simulink model "v1_2025_10_20_D1_first_team_draft"  (R2025a)
settings: Solver=FixedStepAuto  StartTime=0.0  StopTime=10.0  FixedStep=1e-3  RelTol=1e-3  EnableMultiTasking=on
undefined symbols (not defined in the file): D0, D1, D10, D11, D12, D13, D2, D3, D4, D5, D6, D7, D8, D9, PTA0, PTA1, PTA2, PTB23, PTB9, PTC16, PTC17, PTC2, PTC3, PTC4, PTD0, PTD1, PTD2, PTD3
libraries: frdmk64flib x14
settings Model: ExtModeTrigDuration=5  Creator=seohj  LastModifiedBy=seohj
settings OptimizationCC: DefaultParameterBehavior=Inlined  EnhancedBackFolding=on  PassReuseOutputArgsAs=Individual arguments  ZeroExternalMemoryAtStartup=off  ZeroInternalMemoryAtStartup=off  MaxStackSize=64  OptimizeBlockOrder=speed  DifferentSizesBufferReuse=on  OptimizationCustomize=off  EfficientTunableParamExpr=on
settings DebuggingCC: ParameterTunabilityLossMsg=error
settings HardwareCC: ProdBitPerPointer=32.0  ProdBitPerSizeT=32.0  ProdBitPerPtrDiffT=32.0  ProdLargestAtomicInteger=Long  ProdLargestAtomicFloat=Double  ProdWordSize=32.0  ProdHWDeviceType=ARM Compatible->ARM Cortex
settings SFSimCC: MATLABDynamicMemAlloc=off
settings RTWCC: SystemTargetFile=ert.tlc  HardwareBoard=NXP FRDM-K64F  TLCOptions="-aInlineSetEventsForThisBaseRateFcn=TLC_FALSE -aSuppressMultiTaskScheduler=TLC_FALSE  -aRateBasedStepFcn=0"  TemplateMakefile=ert_default_tmf  Toolchain=GNU Tools for ARM Embedded Processors  Description=Embedded Coder
settings CodeAppCC: ForceParamTrailComments=on  IgnoreCustomStorageClasses=off  OperatorAnnotations=on  SimulinkDataObjDesc=on  SFDataObjDesc=on  InsertBlockDesc=on
settings ERTTargetCC: ExtModeTransport=4.0  ExtModeStaticAlloc=off  ExtModeMexFile=sendToCommService  ExtModeIntrfLevel=Level1

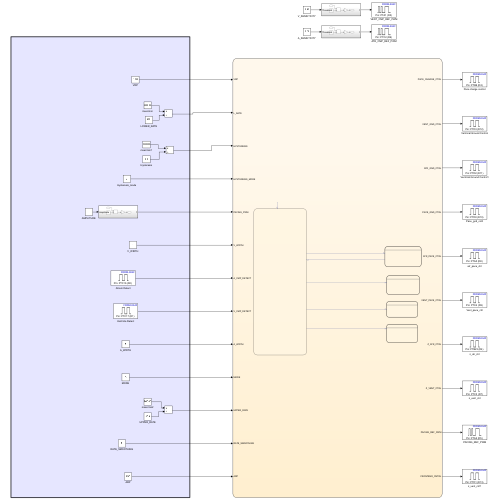
[thumbnail: Simulink's stored preview of the top-level diagram]
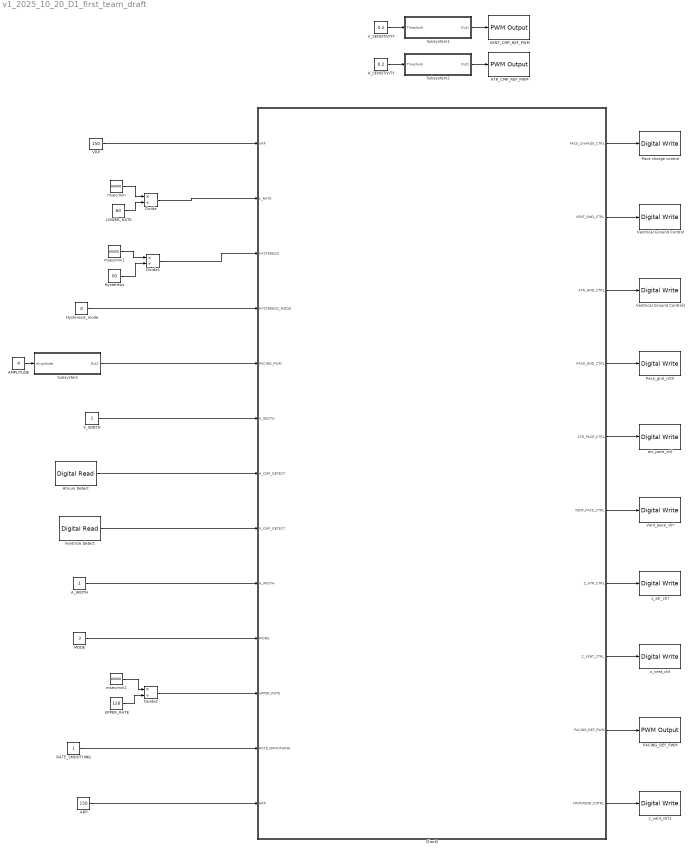
== system v1_2025_10_20_D1_first_team_draft ==
  AMPLITUDE : Constant  Value=4  OutDataTypeStr=int16
  ARP : Constant  Value=150  OutDataTypeStr=int16
  ATR_CMP_REF_PWM : frdmk64flib/PWM Output  Whichpin=PTC2 (D6)  InitialFrequency=2000  InitialDutyCycle=0
  A_SENSITIVITY : Constant  Value=0.2  OutDataTypeStr=double
  A_WIDTH : Constant  OutDataTypeStr=int16
  Atrium Detect : frdmk64flib/Digital Read  Whichpin=PTC16 (D0)  SampleTime=-1
  Chart2 : Stateflow chart  TreatAsAtomicUnit=on
      settings: PortSchema="{\"entries\":[{\"content\":{\"sides\":[{\"content\":{\"connectorIds\":[\"In1\",\"In8\",\"In3\",\"In4\",\"In5\",\"In9\",\"In10\",\"In11\",\"In12\",\"In6\",\"In13\",\"In7\",\"In2\"]},\"type\":\"ConnectorPlacement.EquallySpacedRectSide\",\"uuid\":\"eb0c691f-8d42-442e-bcbf-fb5e5d0eed13\"},{\"content\":{\"connectorIds\":[\"Out1\",\"Out2\",\"Out3\",\"Out4\",\"Out5\",\"Out6\",\"Out7\",\"Out8\",\"Out9\",\"Out10\"],\"side\":\"RIGHT\"},\"type\":\"ConnectorPlacement.EquallySpacedRectSide\",\"uuid\":\"51fddc5a-1884-4d13-98b7-b2e7f62644c5\"},{\"content\":{\"side\":\"TOP\"},\"type\":\"ConnectorPlacement.EquallySpacedRectSide\",\"uuid\":\"c0de6dfc-3a40-48f1-a3e4-7cd76d4b9b4b\"},{\"content\":{\"side\":\"BOTTOM\"},\"type\":\"ConnectorPlacement.EquallySpacedRectSide\",\"uuid\":\"2c1acec7-1ddf-4f64-9578-e80022136ca6\"}]},\"type\":\"ConnectorPlacement.EquallySpacedConnector\",\"uuid\":\"3f5ef44b-ad1c-43dd-8b19-21cef7f1f7f1\"}],\"packageUris\":[\"http://schema.mathworks.com/mf0/Connector/R2020b\"],\"version\":\"1.0\"}"
  Divide : Product  Inputs=*/
  Divide1 : Product  Inputs=*/
  Divide2 : Product  Inputs=*/
  Hysteresis : Constant  Value=50
  Hysteresis_mode : Constant  Value=0
  LOWER_RATE : Constant  Value=60  OutDataTypeStr=int16
  MODE : Constant  Value=3  OutDataTypeStr=int16
  PACING_REF_PWM : frdmk64flib/PWM Output  Whichpin=PTA2 (D5)  InitialFrequency=2000  InitialDutyCycle=0
  Pace charge control : frdmk64flib/Digital Write  Whichpin=PTB9 (D2)
  Pace_gnd_cntrl : frdmk64flib/Digital Write  Whichpin=PTD0 (D10)
  RATE_SMOOTHING : Constant  OutDataTypeStr=int16
  Subsystem : Subsystem
  Subsystem1 : Subsystem
  Subsystem2 : Subsystem
  UPPER_RATE : Constant  Value=128  OutDataTypeStr=int16
  VENT_CMP_REF_PWM : frdmk64flib/PWM Output  Whichpin=PTA1 (D3)  InitialFrequency=2000  InitialDutyCycle=0
  VRP : Constant  Value=150  OutDataTypeStr=int16
  V_SENSITIVITY : Constant  Value=0.2  OutDataTypeStr=double
  V_WIDTH : Constant  OutDataTypeStr=int16
  Vent_pace_ctrl : frdmk64flib/Digital Write  Whichpin=PTC4 (D9)
  Ventrical Ground Control : frdmk64flib/Digital Write  Whichpin=PTD3 (D12)
  Ventrical Ground Control1 : frdmk64flib/Digital Write  Whichpin=PTD2 (D11)
  Ventricle Detect : frdmk64flib/Digital Read  Whichpin=PTC17 (D1)  SampleTime=-1
  atr_pace_ctrl : frdmk64flib/Digital Write  Whichpin=PTA0 (D8)
  msec/min : Constant  Value=60000  OutDataTypeStr=double  LockScale=on
  msec/min1 : Constant  Value=60000  OutDataTypeStr=double  LockScale=on
  msec/min2 : Constant  Value=60000  OutDataTypeStr=double  LockScale=on
  z_atr_ctrl : frdmk64flib/Digital Write  Whichpin=PTB23 (D4)
  z_vent_ctrl : frdmk64flib/Digital Write  Whichpin=PTC3 (D7)
  z_vent_ctrl1 : frdmk64flib/Digital Write  Whichpin=PTD1 (D13)
  wires:
  A_WIDTH/1 -> Chart2/12(A_WIDTH)
  V_WIDTH/1 -> Chart2/9(V_WIDTH)
  Ventricle Detect/1 -> Chart2/11(V_CMP_DETECT)
  RATE_SMOOTHING/1 -> Chart2/7(RATE_SMOOTHING)
  VRP/1 -> Chart2/1(VRP)
  ARP/1 -> Chart2/2(ARP)
  MODE/1 -> Chart2/6(MODE)
  Atrium Detect/1 -> Chart2/10(A_CMP_DETECT)
  msec/min/1 -> Divide/1
  LOWER_RATE/1 -> Divide/2
  Divide/1 -> Chart2/8(L_RATE)
  msec/min1/1 -> Divide1/1
  Divide1/1 -> Chart2/3(HYSTERESIS)
  msec/min2/1 -> Divide2/1
  Divide2/1 -> Chart2/13(UPPER_RATE)
  UPPER_RATE/1 -> Divide2/2
  Chart2/1(PACE_CHARGE_CTRL) -> Pace charge control/1
  Chart2/2(VENT_GND_CTRL) -> Ventrical Ground Control/1
  Chart2/3(ATR_GND_CTRL) -> Ventrical Ground Control1/1
  Chart2/7(Z_ATR_CTRL) -> z_atr_ctrl/1
  Chart2/8(Z_VENT_CTRL) -> z_vent_ctrl/1
  Chart2/6(VENT_PACE_CTRL) -> Vent_pace_ctrl/1
  Chart2/5(ATR_PACE_CTRL) -> atr_pace_ctrl/1
  Chart2/4(PACE_GND_CTRL) -> Pace_gnd_cntrl/1
  Chart2/9(PACING_REF_PWM) -> PACING_REF_PWM/1
  AMPLITUDE/1 -> Subsystem/1(Amplitude)
  Subsystem/1(Out1) -> Chart2/5(PACING_PWM)
  Subsystem1/1(Out1) -> VENT_CMP_REF_PWM/1
  V_SENSITIVITY/1 -> Subsystem1/1(Threshold)
  Subsystem2/1(Out1) -> ATR_CMP_REF_PWM/1
  A_SENSITIVITY/1 -> Subsystem2/1(Threshold)
  Hysteresis/1 -> Divide1/2
  Hysteresis_mode/1 -> Chart2/4(HYSTERESIS_MODE)
  Chart2/10(FRONTEND_CNTRL) -> z_vent_ctrl1/1

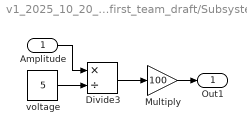
== system v1_2025_10_20_D1_first_team_draft/Subsystem ==
  Amplitude : Inport
  Divide3 : Product  Inputs=*/
  Multiply : Gain  Gain=100
  voltage : Constant  Value=5  OutDataTypeStr=int16
  Out1 : Outport
  wires:
  Divide3/1 -> Multiply/1
  Multiply/1 -> Out1/1
  voltage/1 -> Divide3/2
  Amplitude/1 -> Divide3/1

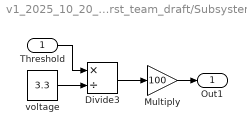
== system v1_2025_10_20_D1_first_team_draft/Subsystem1 ==
  Threshold : Inport
  Divide3 : Product  Inputs=*/
  Multiply : Gain  Gain=100
  voltage : Constant  Value=3.3  OutDataTypeStr=double
  Out1 : Outport
  wires:
  Divide3/1 -> Multiply/1
  Multiply/1 -> Out1/1
  voltage/1 -> Divide3/2
  Threshold/1 -> Divide3/1

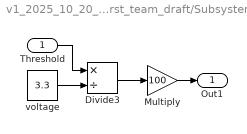
== system v1_2025_10_20_D1_first_team_draft/Subsystem2 ==
  Threshold : Inport
  Divide3 : Product  Inputs=*/
  Multiply : Gain  Gain=100
  voltage : Constant  Value=3.3  OutDataTypeStr=double
  Out1 : Outport
  wires:
  Divide3/1 -> Multiply/1
  Multiply/1 -> Out1/1
  voltage/1 -> Divide3/2
  Threshold/1 -> Divide3/1

== stateflow chart v1_2025_10_20_D1_first_team_draft/Chart2 ==
  state START
  state AOO
    state AOO
      entry:
      %Charge Capacitor
      PACING_REF_PWM = PACING_PWM
      ATR_PACE_CTRL = LOW
      VENT_PACE_CTRL = LOW
      PACE_CHARGE_CTRL = HIGH
      %Discharge Blocking Capactior
      PACE_GND_CTRL = HIGH
      VENT_PACE_CTRL = LOW
      Z_ATR_CTRL = LOW
      Z_VENT_CTRL = LOW
      ATR_PACE_CTRL = LOW
      ATR_GND_CTRL = HIGH
      VENT_GND_CTRL = LOW
    state AOO_PULSE
      entry:
      %Begin discharging C22 and charging C21
      PACE_CHARGE_CTRL= LOW
      PACE_GND_CTRL = HIGH
      ATR_PACE_CTRL = HIGH
      ATR_GND_CTRL = LOW
      Z_ATR_CTRL = LOW
      Z_VENT_CTRL = LOW
      VENT_GND_CTRL = LOW
      VENT_PACE_CTRL = LOW
    (default) -> AOO.AOO
    AOO.AOO -> AOO_PULSE : [after(L_RATE - A_WIDTH,msec)]
    AOO_PULSE -> AOO.AOO : [after(A_WIDTH,msec)]
  state VOO
    state VOO
      entry:
      %Charge Capacitor C22
      ATR_PACE_CTRL = LOW
      VENT_PACE_CTRL = LOW
      PACING_REF_PWM = PACING_PWM
      PACE_CHARGE_CTRL = HIGH
      %Discharge Blocking Capacitor
      VENT_PACE_CTRL = LOW
      PACE_GND_CTRL = HIGH
      ATR_PACE_CTRL = LOW
      ATR_GND_CTRL = LOW
      Z_ATR_CTRL = LOW
      Z_VENT_CTRL = LOW
      VENT_GND_CTRL = HIGH
    state VOO_PULSE
      entry:
      %Begin discharging C22 and charging C21
      PACE_CHARGE_CTRL= LOW
      PACE_GND_CTRL = HIGH
      ATR_PACE_CTRL = LOW
      ATR_GND_CTRL = LOW
      Z_ATR_CTRL = LOW
      Z_VENT_CTRL = LOW
      VENT_GND_CTRL = LOW
      VENT_PACE_CTRL = HIGH
    (default) -> VOO.VOO
    VOO.VOO -> VOO_PULSE : [after(L_RATE - V_WIDTH,msec)]
    VOO_PULSE -> VOO.VOO : [after(V_WIDTH,msec)]
  state AAI
    state AAI
      entry:
      %Charge Capacitor
      PACING_REF_PWM = PACING_PWM
      ATR_PACE_CTRL = LOW
      VENT_PACE_CTRL = LOW
      PACE_CHARGE_CTRL = HIGH
      %Discharge Blocking Capactior
      PACE_GND_CTRL = HIGH
      VENT_PACE_CTRL = LOW
      Z_ATR_CTRL = LOW
      Z_VENT_CTRL = LOW
      ATR_PACE_CTRL = LOW
      ATR_GND_CTRL = HIGH
      VENT_GND_CTRL = LOW
      FRONTEND_CNTRL = HIGH
    state AAI_PULSE
      entry:
      %Begin discharging C22 and charging C21
      PACE_CHARGE_CTRL= LOW
      PACE_GND_CTRL = HIGH
      ATR_PACE_CTRL = HIGH
      ATR_GND_CTRL = LOW
      Z_ATR_CTRL = LOW
      Z_VENT_CTRL = LOW
      VENT_GND_CTRL = LOW
      VENT_PACE_CTRL = LOW
      FRONTEND_CNTRL = LOW
    state Buffer
    state AAI_ARP
      entry:
      %Charge Capacitor
      PACING_REF_PWM = PACING_PWM
      ATR_PACE_CTRL = LOW
      VENT_PACE_CTRL = LOW
      PACE_CHARGE_CTRL = LOW
      %Discharge Blocking Capactior
      PACE_GND_CTRL = HIGH
      VENT_PACE_CTRL = LOW
      Z_ATR_CTRL = LOW
      Z_VENT_CTRL = LOW
      ATR_PACE_CTRL = LOW
      ATR_GND_CTRL = HIGH
      VENT_GND_CTRL = LOW
      FRONTEND_CNTRL = LOW
    AAI.AAI -> AAI_PULSE [order 2] : [after(HYSTERESIS - A_WIDTH-ARP,msec) & HYSTERESIS_MODE == 1]
    (default) -> AAI.AAI
    AAI.AAI -> AAI_PULSE [order 3] : [after(L_RATE - A_WIDTH-ARP,msec) & HYSTERESIS_MODE == 0 ]
    AAI.Buffer -> AAI.Buffer [order 2] : [A_CMP_DETECT == HIGH]
    AAI.AAI -> AAI.Buffer [order 1] : [A_CMP_DETECT == HIGH]
    AAI.Buffer -> AAI.AAI [order 3] : [after(HYSTERESIS,msec) & HYSTERESIS_MODE ==1]
    AAI.Buffer -> AAI.AAI [order 1] : [after(L_RATE,msec) & HYSTERESIS_MODE == 0]
    AAI_PULSE -> AAI_ARP : [after(A_WIDTH,msec)]
    AAI_ARP -> AAI.AAI : [after(ARP,msec)]
  state VVI
    state VVI
      entry:
      %Charge Capacitor C22
      ATR_PACE_CTRL = LOW
      VENT_PACE_CTRL = LOW
      PACING_REF_PWM = PACING_PWM
      PACE_CHARGE_CTRL = HIGH
      %Discharge Blocking Capacitor
      VENT_PACE_CTRL = LOW
      PACE_GND_CTRL = HIGH
      ATR_PACE_CTRL = LOW
      ATR_GND_CTRL = LOW
      Z_ATR_CTRL = LOW
      Z_VENT_CTRL = LOW
      VENT_GND_CTRL = HIGH
      FRONTEND_CNTRL = HIGH
    state VVI_PULSE
      entry:
      %Begin discharging C22 and charging C21
      PACE_CHARGE_CTRL= LOW
      PACE_GND_CTRL = HIGH
      ATR_PACE_CTRL = LOW
      ATR_GND_CTRL = LOW
      Z_ATR_CTRL = LOW
      Z_VENT_CTRL = LOW
      VENT_GND_CTRL = LOW
      VENT_PACE_CTRL = HIGH
      FRONTEND_CNTRL = LOW
    state Buffer
    state VVI_VRP
      entry:
      %Charge Capacitor C22
      ATR_PACE_CTRL = LOW
      VENT_PACE_CTRL = LOW
      PACING_REF_PWM = PACING_PWM
      PACE_CHARGE_CTRL = LOW
      %Discharge Blocking Capacitor
      VENT_PACE_CTRL = LOW
      PACE_GND_CTRL = HIGH
      ATR_PACE_CTRL = LOW
      ATR_GND_CTRL = LOW
      Z_ATR_CTRL = LOW
      Z_VENT_CTRL = LOW
      VENT_GND_CTRL = HIGH
      FRONTEND_CNTRL = LOW
    VVI.VVI -> VVI_PULSE [order 3] : [after(HYSTERESIS - A_WIDTH-ARP,msec) & HYSTERESIS_MODE==1 ]
    (default) -> VVI.VVI
    VVI.VVI -> VVI_PULSE [order 1] : [after(L_RATE - V_WIDTH-VRP,msec) & HYSTERESIS_MODE == 0 ]
    VVI.Buffer -> VVI.Buffer [order 2] : [V_CMP_DETECT == HIGH]
    VVI.VVI -> VVI.Buffer [order 2] : [V_CMP_DETECT == HIGH]
    VVI.Buffer -> VVI.VVI [order 3] : [after(HYSTERESIS,msec) & HYSTERESIS_MODE ==1]
    VVI.Buffer -> VVI.VVI [order 1] : [after(L_RATE,msec)]
    VVI_PULSE -> VVI_VRP : [after(V_WIDTH,msec)]
    VVI_VRP -> VVI.VVI : [after(VRP,msec)]
  (default) -> START
  START -> AOO [order 1] : [MODE ==1]
  AOO -> START : [MODE ~=1]
  START -> VOO [order 2] : [MODE ==2]
  START -> AAI [order 3] : [MODE==3]
  START -> VVI [order 4] : [MODE ==4]
  data: VRP input; ARP input; HYSTERESIS input; HYSTERESIS_MODE input; PACING_PWM input; MODE input; RATE_SMOOTHING input; L_RATE input; V_WIDTH input; A_CMP_DETECT input; V_CMP_DETECT input; A_WIDTH input; UPPER_RATE input; PACE_CHARGE_CTRL output; VENT_GND_CTRL output; ATR_GND_CTRL output; PACE_GND_CTRL output; ATR_PACE_CTRL output; VENT_PACE_CTRL output; Z_ATR_CTRL output; Z_VENT_CTRL output; HIGH local boolean =true; LOW local boolean =false; PACING_REF_PWM output; FRONTEND_CNTRL output
